simulink model "STM_Propagator"  (R2024b)
settings: Solver=ode4  StartTime=0.0  StopTime=TSim  FixedStep=1e-1  RelTol=1e-3
model workspace (MAT data in the model file):
  BVH_bboxMax = Simulink.Parameter
  BVH_bboxMax.Value = [284.93805 4.355131 284.93805 278.0491 284.93805 284.65656 284.93805 139.47609 284.93805 284.93805 268.4671 268.4671 ... (24573 elements, 8191x3)]
  BVH_bboxMax.Complexity = 'real'
  BVH_bboxMax.Dimensions = [8191 3]
  BVH_bboxMax.DataType = 'auto'
  BVH_bboxMin = Simulink.Parameter
  BVH_bboxMin.Value = [-277.88974 -277.88974 -8.175628 -8.175628 -7.5725703 -7.2454505 -7.5725703 -7.5725703 128.49397 129.55234 128.49397 128.49397 ... (24573 elements, 8191x3)]
  BVH_bboxMin.Complexity = 'real'
  BVH_bboxMin.Dimensions = [8191 3]
  BVH_bboxMin.DataType = 'auto'
  BVH_fCount = Simulink.Parameter
  BVH_fCount.Value = [0 0 0 0 0 0 0 0 0 0 0 0 ... (8191 elements, 8191x1)]
  BVH_fCount.Complexity = 'real'
  BVH_fCount.Dimensions = [8191 1]
  BVH_fCount.DataType = 'int32'
  BVH_fStart = Simulink.Parameter
  BVH_fStart.Value = [0 0 0 0 0 0 0 0 0 0 0 0 ... (8191 elements, 8191x1)]
  BVH_fStart.Complexity = 'real'
  BVH_fStart.Dimensions = [8191 1]
  BVH_fStart.DataType = 'int32'
  BVH_faces = Simulink.Parameter
  BVH_faces.Value = [6744 6709 6709 6698 6730 6729 6745 6681 6682 6684 6684 6682 ... (74994 elements, 24998x3)]
  BVH_faces.Complexity = 'real'
  BVH_faces.Dimensions = [24998 3]
  BVH_faces.DataType = 'int32'
  BVH_left = Simulink.Parameter
  BVH_left.Value = [2 4098 4 2052 6 1030 8 520 10 266 12 140 ... (8191 elements, 8191x1)]
  BVH_left.Complexity = 'real'
  BVH_left.Dimensions = [8191 1]
  BVH_left.DataType = 'int32'
  BVH_normals = Simulink.Parameter
  BVH_normals.Value = [1 1 1 1 1 1 0 1 1 1 1 1 ... (74994 elements, 24998x3)]
  BVH_normals.Complexity = 'real'
  BVH_normals.Dimensions = [24998 3]
  BVH_normals.DataType = 'auto'
  BVH_right = Simulink.Parameter
  BVH_right.Value = [3 4099 5 2053 7 1031 9 521 11 267 13 141 ... (8191 elements, 8191x1)]
  BVH_right.Complexity = 'real'
  BVH_right.Dimensions = [8191 1]
  BVH_right.DataType = 'int32'
  BVH_vertexList = Simulink.Parameter
  BVH_vertexList.Value = [-118.90262 -122.20188 -116.06995 -125.190315 -127.74983 -122.412506 -131.21611 -134.88121 -129.40932 -138.59775 -133.93816 -136.61743 ... (37503 elements, 12501x3)]
  BVH_vertexList.Complexity = 'real'
  BVH_vertexList.Dimensions = [12501 3]
  BVH_vertexList.DataType = 'auto'
undefined symbols (not defined in the file): environment, gravGrad, init
settings Model: SimulationMode=accelerator  Creator=pierb  LastModifiedBy=pierb

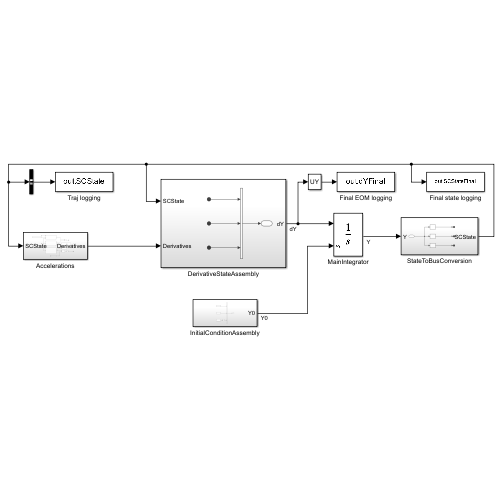
[thumbnail: Simulink's stored preview of the top-level diagram]
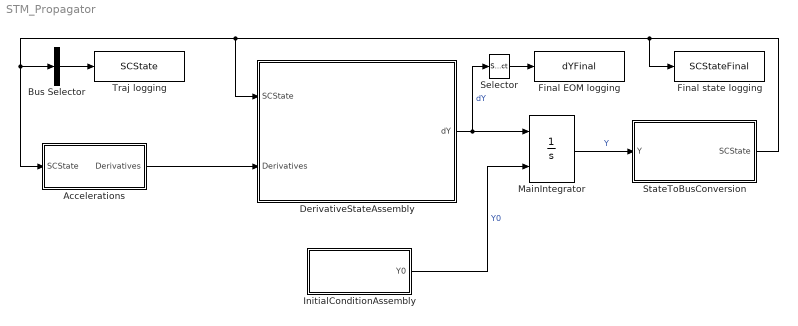
== system STM_Propagator ==
  Accelerations : Subsystem
  Bus Selector : BusSelector  OutputSignals=position,velocity  OutputAsBus=on
  DerivativeStateAssembly : Subsystem
  Final EOM logging : ToWorkspace  VariableName=dYFinal  SampleTime=-1
      settings: MaxDataPoints=1
  Final state logging : ToWorkspace  VariableName=SCStateFinal  SampleTime=-1
      settings: MaxDataPoints=1
  InitialConditionAssembly : Subsystem
  MainIntegrator : Integrator  InitialConditionSource=external
  Selector : Selector  InputPortWidth=42  IndexOptions=Index vector (dialog)  Indices=1:6  OutputSizes=1
  StateToBusConversion : Subsystem
  Traj logging : ToWorkspace  VariableName=SCState  SaveFormat=Timeseries  SampleTime=-1
  wires:
  DerivativeStateAssembly/1(dY) -> Selector/1, MainIntegrator/1  "dY"
  InitialConditionAssembly/1(Y0) -> MainIntegrator/2  "Y0"
  MainIntegrator/1 -> StateToBusConversion/1(Y)  "Y"
  StateToBusConversion/1(SCState) -> Accelerations/1(SCState), Bus Selector/1, DerivativeStateAssembly/1(SCState), Final state logging/1
  Accelerations/1(Derivatives) -> DerivativeStateAssembly/2(Derivatives)
  Bus Selector/1 -> Traj logging/1
  Selector/1 -> Final EOM logging/1

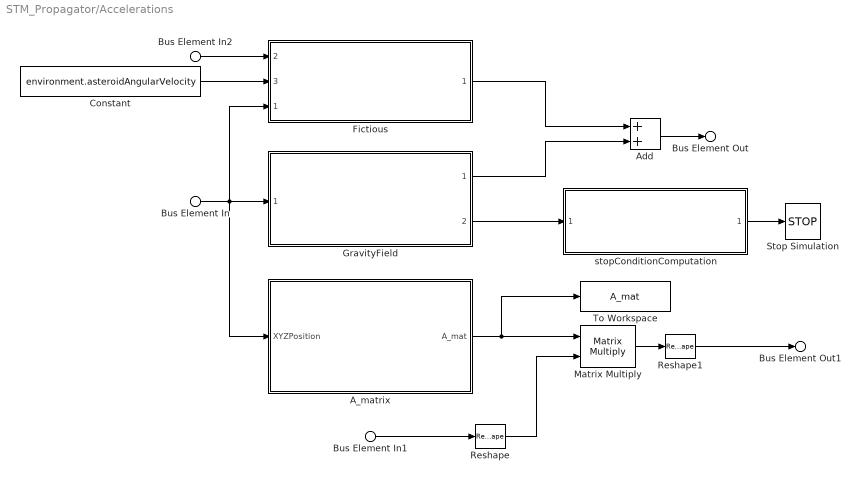
== system STM_Propagator/Accelerations ==
  Bus Element In : Inport  PortName=SCState  Element=position
  Bus Element In2 : Inport  PortName=SCState  Element=velocity
  Bus Element In1 : Inport  PortName=SCState  Element=STM
  A_matrix : Subsystem
  Add : Sum
  Constant : Constant  Value=environment.asteroidAngularVelocity
  Fictious : Subsystem  ReferencedSubsystem=Fictious
      settings: PortSchema="{\"entries\":[{\"content\":{\"sides\":[{\"content\":{\"connectorIds\":[\"In2\",\"In3\",\"In1\"]},\"type\":\"ConnectorPlacement.EquallySpacedRectSide\",\"uuid\":\"a3b8630a-6c78-4619-a2af-aa515379054c\"},{\"content\":{\"connectorIds\":[\"Out1\"],\"side\":\"RIGHT\"},\"type\":\"ConnectorPlacement.EquallySpacedRectSide\",\"uuid\":\"d9fece68-8f84-49ee-b4a5-ef42046b02f8\"},{\"content\":{\"side\":\"TOP\"},\"type\":\"ConnectorPlacement.EquallySpacedRectSide\",\"uuid\":\"cc219af0-ea4f-4bce-8591-fe8fb94efc15\"}]},\"type\":\"ConnectorPlacement.EquallySpacedConnector\",\"uuid\":\"d534c14c-16b8-460a-b930-b163aa0cf1f7\"}],\"packageUris\":[\"http://schema.mathworks.com/mf0/Connector/R2020b\"],\"version\":\"1.0\"}"
  GravityField : Subsystem  ReferencedSubsystem=GravityField
  Matrix Multiply : Product  Multiplication=Matrix(*)
  Reshape : Reshape  OutputDimensionality=Customize  OutputDimensions=[6,6]
  Reshape1 : Reshape  OutputDimensions=[6,6]
  Stop Simulation : Stop
  To Workspace : ToWorkspace  VariableName=A_mat  SaveFormat=Timeseries  SampleTime=-1
      settings: MaxDataPoints=Inf
  stopConditionComputation : Subsystem  ReferencedSubsystem=laplaceStopConditionComputation
  Bus Element Out : Outport  PortName=Derivatives  Element=dVel
  Bus Element Out1 : Outport  PortName=Derivatives  Element=dSTM
  wires:
  Bus Element In/1 -> A_matrix/1(XYZPosition), GravityField/1, Fictious/1
  Bus Element In2/1 -> Fictious/2
  Constant/1 -> Fictious/3
  Add/1 -> Bus Element Out/1
  Fictious/1 -> Add/1
  GravityField/2 -> stopConditionComputation/1
  stopConditionComputation/1 -> Stop Simulation/1
  GravityField/1 -> Add/2
  Reshape1/1 -> Bus Element Out1/1
  Bus Element In1/1 -> Reshape/1
  A_matrix/1(A_mat) -> To Workspace/1, Matrix Multiply/1
  Reshape/1 -> Matrix Multiply/2
  Matrix Multiply/1 -> Reshape1/1

== system STM_Propagator/DerivativeStateAssembly ==
  Bus Element In2 : Inport  PortName=SCState  Element=velocity
  Bus Element In1 : Inport  Port=2  PortName=Derivatives  Element=dVel
  Bus Element In : Inport  Port=2  PortName=Derivatives  Element=dSTM
  Vector Concatenate : Concatenate  NumInputs=3
  dY : Outport
  wires:
  Vector Concatenate/1 -> dY/1
  Bus Element In/1 -> Vector Concatenate/3
  Bus Element In2/1 -> Vector Concatenate/1
  Bus Element In1/1 -> Vector Concatenate/2

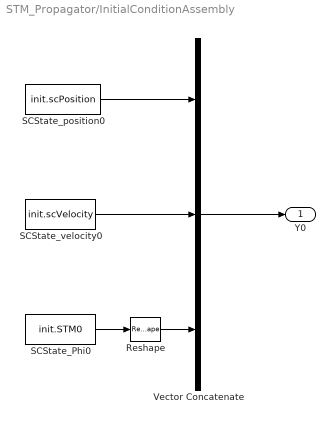
== system STM_Propagator/InitialConditionAssembly ==
  Reshape : Reshape
  SCState_Phi0 : Constant  Value=init.STM0
  SCState_position0 : Constant  Value=init.scPosition
  SCState_velocity0 : Constant  Value=init.scVelocity
  Vector Concatenate : Concatenate  NumInputs=3
  Y0 : Outport
  wires:
  SCState_position0/1 -> Vector Concatenate/1
  Vector Concatenate/1 -> Y0/1
  SCState_velocity0/1 -> Vector Concatenate/2
  SCState_Phi0/1 -> Reshape/1
  Reshape/1 -> Vector Concatenate/3

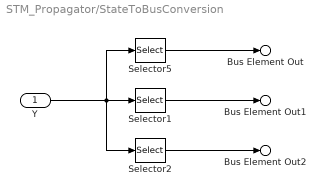
== system STM_Propagator/StateToBusConversion ==
  Y : Inport
  Selector1 : Selector  InputPortWidth=42  IndexOptions=Index vector (dialog)  Indices=[4:6]  OutputSizes=1
  Selector2 : Selector  InputPortWidth=42  IndexOptions=Index vector (dialog)  Indices=[7:42]  OutputSizes=1
  Selector5 : Selector  InputPortWidth=42  IndexOptions=Index vector (dialog)  Indices=[1:3]  OutputSizes=1
  Bus Element Out : Outport  PortName=SCState  Element=position
  Bus Element Out1 : Outport  PortName=SCState  Element=velocity
  Bus Element Out2 : Outport  PortName=SCState  Element=STM
  wires:
  Y/1 -> Selector5/1, Selector2/1, Selector1/1
  Selector5/1 -> Bus Element Out/1
  Selector1/1 -> Bus Element Out1/1
  Selector2/1 -> Bus Element Out2/1

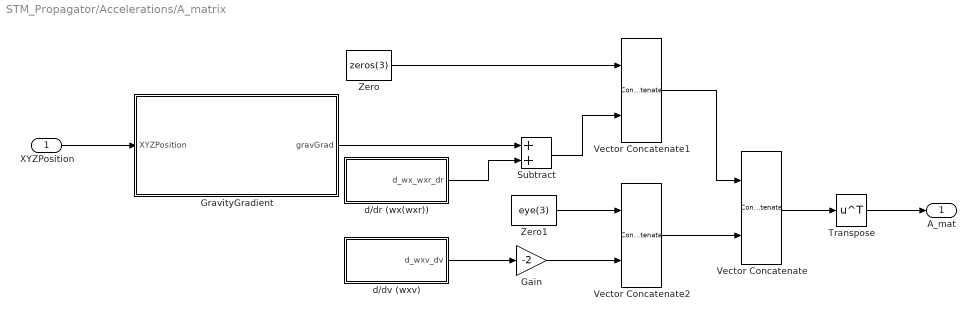
== system STM_Propagator/Accelerations/A_matrix ==
  XYZPosition : Inport
  Gain : Gain  Gain=-2
  GravityGradient : Subsystem
  Subtract : Sum
  Transpose : Math  Operator=transpose
  Vector Concatenate : Concatenate  Mode=Multidimensional array
  Vector Concatenate1 : Concatenate  Mode=Multidimensional array  ConcatenateDimension=2
  Vector Concatenate2 : Concatenate  Mode=Multidimensional array  ConcatenateDimension=2
  Zero : Constant  Value=zeros(3)  OutDataTypeStr=Inherit: Inherit via back propagation
  Zero1 : Constant  Value=eye(3)  OutDataTypeStr=Inherit: Inherit via back propagation
  d/dr (wx(wxr)) : Subsystem
  d/dv (wxv) : Subsystem
  A_mat : Outport
  wires:
  XYZPosition/1 -> GravityGradient/1(XYZPosition)
  Vector Concatenate/1 -> Transpose/1
  Vector Concatenate1/1 -> Vector Concatenate/1
  GravityGradient/1(gravGrad) -> Subtract/1
  Zero/1 -> Vector Concatenate1/1
  d/dr (wx(wxr))/1(d_wx_wxr_dr) -> Subtract/2
  Subtract/1 -> Vector Concatenate1/2
  Vector Concatenate2/1 -> Vector Concatenate/2
  Zero1/1 -> Vector Concatenate2/1
  d/dv (wxv)/1(d_wxv_dv) -> Gain/1
  Gain/1 -> Vector Concatenate2/2
  Transpose/1 -> A_mat/1

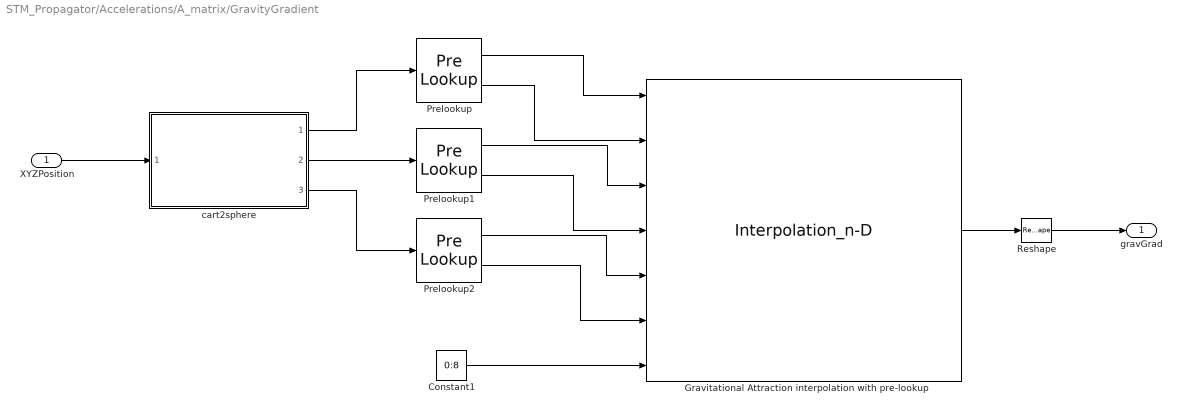
== system STM_Propagator/Accelerations/A_matrix/GravityGradient ==
  XYZPosition : Inport
  Constant1 : Constant  Value=0:8
  Gravitational Attraction interpolation with pre-lookup : Interpolation_n-D  NumberOfTableDimensions=4  Table=reshape(gravGrad, [100 50 100 9])  ExtrapMethod=Clip  NumSelectionDims=1  RndMeth=Simplest
      settings: InputPortMap=u0,u1,u2,u3,u4,u5,u6
  Prelookup : PreLookup  BreakpointsData=environment.asteroidCoords.radius  BeginIndexSearchUsingPreviousIndexResult=on  ExtrapMethod=Linear  RndMeth=Simplest
  Prelookup1 : PreLookup  BreakpointsData=environment.asteroidCoords.polar  IndexSearchMethod=Linear search  BeginIndexSearchUsingPreviousIndexResult=on  DiagnosticForOutOfRangeInput=Warning  RndMeth=Simplest
  Prelookup2 : PreLookup  BreakpointsData=environment.asteroidCoords.azimuth  IndexSearchMethod=Linear search  BeginIndexSearchUsingPreviousIndexResult=on  RndMeth=Simplest
  Reshape : Reshape  OutputDimensionality=Customize  OutputDimensions=[3,3]
  cart2sphere : Subsystem  ReferencedSubsystem=cart2sphere
  gravGrad : Outport
  wires:
  Prelookup2/1 -> Gravitational Attraction interpolation with pre-lookup/5
  Prelookup/2 -> Gravitational Attraction interpolation with pre-lookup/2
  Prelookup1/2 -> Gravitational Attraction interpolation with pre-lookup/4
  cart2sphere/3 -> Prelookup2/1
  cart2sphere/2 -> Prelookup1/1
  Prelookup1/1 -> Gravitational Attraction interpolation with pre-lookup/3
  cart2sphere/1 -> Prelookup/1
  Prelookup/1 -> Gravitational Attraction interpolation with pre-lookup/1
  Prelookup2/2 -> Gravitational Attraction interpolation with pre-lookup/6
  XYZPosition/1 -> cart2sphere/1
  Gravitational Attraction interpolation with pre-lookup/1 -> Reshape/1
  Constant1/1 -> Gravitational Attraction interpolation with pre-lookup/7
  Reshape/1 -> gravGrad/1

== system STM_Propagator/Accelerations/A_matrix/d//dr (wx(wxr)) ==
  Constant : Constant  Value=environment.asteroidAngularVelocity
  Matrix Concatenate : Concatenate  NumInputs=3  Mode=Multidimensional array  ConcatenateDimension=2
  d_drx : Subsystem
  d_dry : Subsystem
  d_drz : Subsystem
  d_wx_wxr_dr : Outport
  wires:
  Matrix Concatenate/1 -> d_wx_wxr_dr/1
  d_drx/1(d_drx) -> Matrix Concatenate/1
  d_drz/1(d_drz) -> Matrix Concatenate/3
  d_dry/1(d_dry) -> Matrix Concatenate/2
  Constant/1 -> d_drz/1(w_vec), d_drx/1(w_vec), d_dry/1(w_vec)

== system STM_Propagator/Accelerations/A_matrix/d//dv (wxv) ==
  Constant : Constant  Value=environment.asteroidAngularVelocity
  Matrix Concatenate : Concatenate  NumInputs=3  Mode=Multidimensional array  ConcatenateDimension=2
  d_dvx : Subsystem
  d_dvy : Subsystem
  d_dvz : Subsystem
  d_wxv_dv : Outport
  wires:
  Constant/1 -> d_dvz/1(w_vec), d_dvy/1(w_vec), d_dvx/1(w_vec)
  d_dvy/1(d_dvy) -> Matrix Concatenate/2
  d_dvz/1(d_dvz) -> Matrix Concatenate/3
  d_dvx/1(d_dvx) -> Matrix Concatenate/1
  Matrix Concatenate/1 -> d_wxv_dv/1

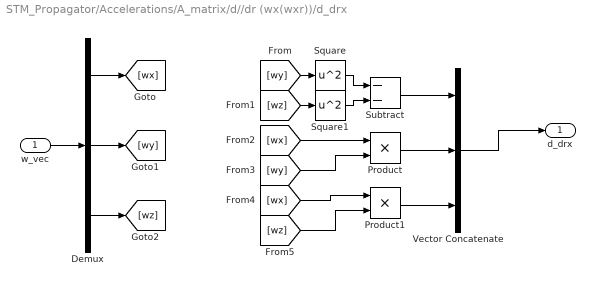
== system STM_Propagator/Accelerations/A_matrix/d//dr (wx(wxr))/d_drx ==
  w_vec : Inport
  Demux : Demux  Outputs=3
  Product : Product
  Product1 : Product
  Square : Math  Operator=square
  Square1 : Math  Operator=square
  Subtract : Sum  Inputs=--
  Vector Concatenate : Concatenate  NumInputs=3
  d_drx : Outport
  wires:
  Subtract/1 -> Vector Concatenate/1
  [wy] -> Product/2
  Square/1 -> Subtract/1
  Square1/1 -> Subtract/2
  [wx] -> Product/1
  Vector Concatenate/1 -> d_drx/1
  [wz] -> Square1/1
  [wy] -> Square/1
  Product/1 -> Vector Concatenate/2
  [wx] -> Product1/1
  [wz] -> Product1/2
  Product1/1 -> Vector Concatenate/3
  Demux/3 -> [wz]
  Demux/1 -> [wx]
  w_vec/1 -> Demux/1
  Demux/2 -> [wy]

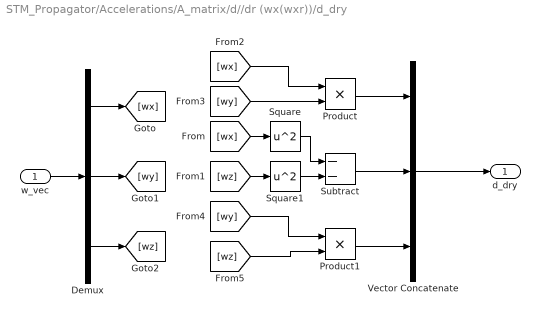
== system STM_Propagator/Accelerations/A_matrix/d//dr (wx(wxr))/d_dry ==
  w_vec : Inport
  Demux : Demux  Outputs=3
  Product : Product
  Product1 : Product
  Square : Math  Operator=square
  Square1 : Math  Operator=square
  Subtract : Sum  Inputs=--
  Vector Concatenate : Concatenate  NumInputs=3
  d_dry : Outport
  wires:
  Product1/1 -> Vector Concatenate/3
  [wz] -> Product1/2
  [wy] -> Product1/1
  Product/1 -> Vector Concatenate/1
  [wx] -> Square/1
  [wz] -> Square1/1
  Vector Concatenate/1 -> d_dry/1
  [wx] -> Product/1
  Square1/1 -> Subtract/2
  Square/1 -> Subtract/1
  [wy] -> Product/2
  Subtract/1 -> Vector Concatenate/2
  Demux/3 -> [wz]
  Demux/2 -> [wy]
  Demux/1 -> [wx]
  w_vec/1 -> Demux/1

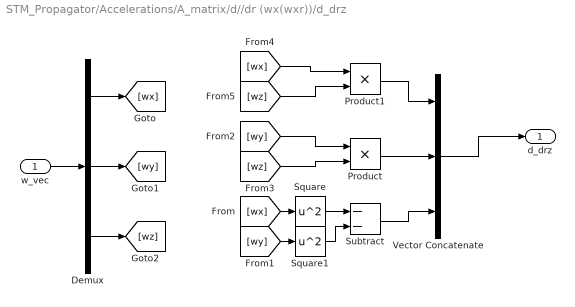
== system STM_Propagator/Accelerations/A_matrix/d//dr (wx(wxr))/d_drz ==
  w_vec : Inport
  Demux : Demux  Outputs=3
  Product : Product
  Product1 : Product
  Square : Math  Operator=square
  Square1 : Math  Operator=square
  Subtract : Sum  Inputs=--
  Vector Concatenate : Concatenate  NumInputs=3
  d_drz : Outport
  wires:
  Subtract/1 -> Vector Concatenate/3
  [wz] -> Product/2
  Square/1 -> Subtract/1
  Square1/1 -> Subtract/2
  [wy] -> Product/1
  Vector Concatenate/1 -> d_drz/1
  [wy] -> Square1/1
  [wx] -> Square/1
  Product/1 -> Vector Concatenate/2
  [wx] -> Product1/1
  [wz] -> Product1/2
  Product1/1 -> Vector Concatenate/1
  Demux/3 -> [wz]
  Demux/2 -> [wy]
  Demux/1 -> [wx]
  w_vec/1 -> Demux/1

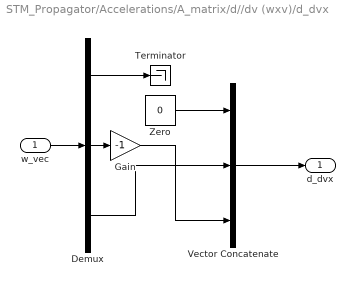
== system STM_Propagator/Accelerations/A_matrix/d//dv (wxv)/d_dvx ==
  w_vec : Inport
  Demux : Demux  Outputs=3
  Gain : Gain  Gain=-1
  Terminator : Terminator
  Vector Concatenate : Concatenate  NumInputs=3
  Zero : Constant  Value=0  OutDataTypeStr=Inherit: Inherit via back propagation
  d_dvx : Outport
  wires:
  w_vec/1 -> Demux/1
  Demux/1 -> Terminator/1
  Demux/2 -> Gain/1
  Demux/3 -> Vector Concatenate/2
  Vector Concatenate/1 -> d_dvx/1
  Zero/1 -> Vector Concatenate/1
  Gain/1 -> Vector Concatenate/3

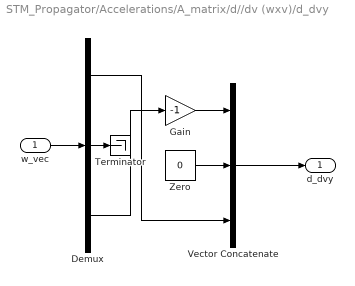
== system STM_Propagator/Accelerations/A_matrix/d//dv (wxv)/d_dvy ==
  w_vec : Inport
  Demux : Demux  Outputs=3
  Gain : Gain  Gain=-1
  Terminator : Terminator
  Vector Concatenate : Concatenate  NumInputs=3
  Zero : Constant  Value=0  OutDataTypeStr=Inherit: Inherit via back propagation
  d_dvy : Outport
  wires:
  Demux/3 -> Gain/1
  Vector Concatenate/1 -> d_dvy/1
  Demux/1 -> Vector Concatenate/3
  w_vec/1 -> Demux/1
  Zero/1 -> Vector Concatenate/2
  Demux/2 -> Terminator/1
  Gain/1 -> Vector Concatenate/1

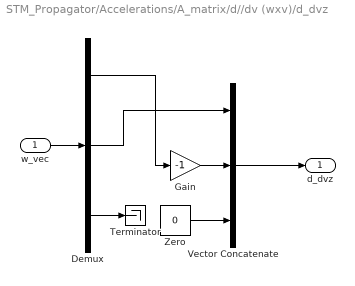
== system STM_Propagator/Accelerations/A_matrix/d//dv (wxv)/d_dvz ==
  w_vec : Inport
  Demux : Demux  Outputs=3
  Gain : Gain  Gain=-1
  Terminator : Terminator
  Vector Concatenate : Concatenate  NumInputs=3
  Zero : Constant  Value=0  OutDataTypeStr=Inherit: Inherit via back propagation
  d_dvz : Outport
  wires:
  Vector Concatenate/1 -> d_dvz/1
  w_vec/1 -> Demux/1
  Demux/1 -> Gain/1
  Demux/2 -> Vector Concatenate/1
  Demux/3 -> Terminator/1
  Zero/1 -> Vector Concatenate/3
  Gain/1 -> Vector Concatenate/2
